simulink model "closedmodel"  (R2024b)
settings: Solver=ode4  StartTime=0.0  StopTime=10  FixedStep=0.001  RelTol=1e-3
values from neighbouring files (symbols this model uses):
  A = 0.00442    [closedparameters.m]
  Af = 0.003689    [closedparameters.m]
  alim = deg2rad(800)    [closedparameters.m]
  b = 0.14    [closedparameters.m]
  bt = 1    [closedparameters.m]
  Cd0 = 0.7    [closedparameters.m]
  Cla = 2    [closedparameters.m]
  Clp = -0.5    [closedparameters.m]
  Cmq = -40    [closedparameters.m]
  CNa = 20    [closedparameters.m]
  Cnr = -40    [closedparameters.m]
  Dgain = 0.2    [closedparameters.m]
  Dgainphi = 0.01    [closedparameters.m]
  dmdt = -(mf - me)/bt    (= -0.063)    [closedparameters.m]
  fin_positions = [dfins 0 fr; dfins -fr 0; dfins 0 -fr; dfins fr 0]    [closedparameters.m]
  gravity = [-9.819 0 0]'    [closedparameters.m]
  Igain = 0    [closedparameters.m]
  Igainphi = 0    [closedparameters.m]
  L = 1.15    [closedparameters.m]
  me = 0.894    [closedparameters.m]
  mf = 0.957    [closedparameters.m]
  N = [0 -1 0; 0 0 -1; 0 1 0; 0 0 1]    [closedparameters.m]
  Pgainphi = deg2rad(10)/ref_phi    [closedparameters.m]
  Pgainy = deg2rad(20)    [closedparameters.m]
  Pgainz = deg2rad(20)    [closedparameters.m]
  r_cp = [Cp 0 0]'    [closedparameters.m]
  ref_phi = pi/2    (= 1.57079632679)    [closedparameters.m]
  refy = 50    [closedparameters.m]
  refz = 50    [closedparameters.m]
  rho = 1.225    [closedparameters.m]
  si = [0 0 1; 0 -1 0; 0 0 -1; 0 1 0]    [closedparameters.m]
  tau = 0.05    [closedparameters.m]
  Vsafe = 0.1    [closedparameters.m]
  wind = [0 10 7]'    [closedparameters.m]
undefined symbols (not defined in the file or in its folder): fin_angles
libraries: slpidlib x5, aerolibanim x1, simulink x1, shared6dof x1, matrix_library x1
settings Model: Creator=tanel  LastModifiedBy=tanel
settings DataIOCC: ReturnWorkspaceOutputs=off

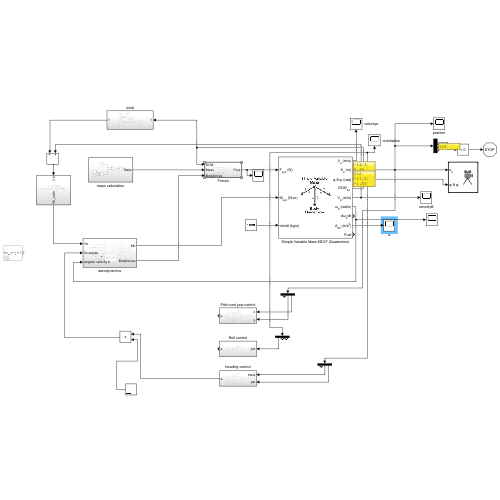
[thumbnail: Simulink's stored preview of the top-level diagram]
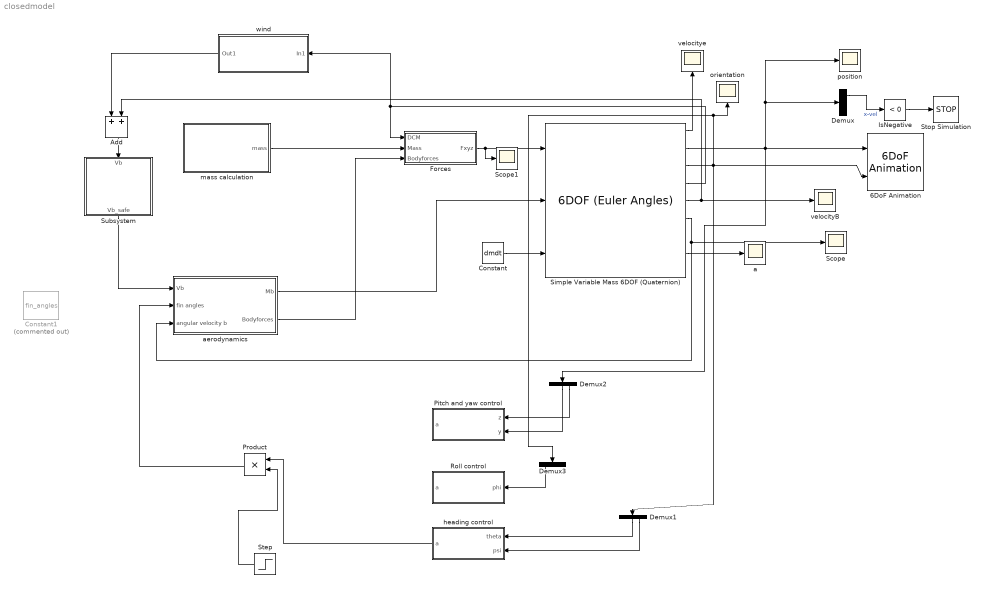
== system closedmodel ==
  6DoF Animation : aerolibanim/6DoF Animation  u1=[0 1000 0 100 0 100]  u2=0.01  u3=1  u4=[400 100 -500]  u5=Fly alongside  u6=[0 15 10]  u7=5  u8=on
  Add : Sum
  Constant : Constant  Value=dmdt
  Constant1 : Constant  Commented=on  Value=fin_angles
  Demux{,1..3} (4 alike) : Demux  Outputs=3
  Forces : Subsystem
  IsNegative : simulink/Logic and Bit Operations/Compare To Zero  relop=<  OutDataTypeStr=boolean
      settings: LibrarySourceBlock=|
      | simulink/Quick Insert/Logic and Bit
      | Operations/IsNegative
  Pitch and yaw control : Subsystem
  Product : Product
  Roll control : Subsystem
  Scope : Scope
  Scope1 : Scope
  Simple Variable Mass 6DOF (Quaternion) : shared6dof/6DOF (Euler Angles)  units=Metric (MKS)  mtype=Simple Variable  rep=Quaternion  xme_0=[0 50 50]  Vm_0=[0 0 0]  eul_0=[0 0 0]  pm_0=[0 0 0]  mass_0=mf  mass_e=me  mass_f=mf  inertia=eye(3)  inertia_e=Ie  inertia_f=If  k_quat=1.0  vre_flag=off  abi_flag=off  aMode=0  xme_statename=''  Vm_statename=''  eul_statename=''  quat_statename=''  pm_statename=''  mass_statename=''
      settings: LibrarySourceBlock=aerolib6dof2/Custom Variable Mass 6DOF (Euler Angles)
  Step : Step  SampleTime=0
  Stop Simulation : Stop
  Subsystem : Subsystem
  a : Scope
  aerodynamics : Subsystem
  heading control : Subsystem
  mass calculation : Subsystem
  orientation : Scope
  position : Scope
  velocityB : Scope
  velocitye : Scope
  wind : Subsystem
  wires:
  Constant/1 -> Simple Variable Mass 6DOF (Quaternion)/3
  Simple Variable Mass 6DOF (Quaternion)/4 -> wind/1(In1), Forces/1(DCM)
  Simple Variable Mass 6DOF (Quaternion)/5 -> Add/2, velocityB/1
  Forces/1(Fxyz) -> Scope1/1, Simple Variable Mass 6DOF (Quaternion)/1
  aerodynamics/1(Mb) -> Simple Variable Mass 6DOF (Quaternion)/2
  Simple Variable Mass 6DOF (Quaternion)/3 -> Demux1/1, 6DoF Animation/2, orientation/1, Demux3/1
  Simple Variable Mass 6DOF (Quaternion)/2 -> Demux/1, position/1, Demux2/1, 6DoF Animation/1
  IsNegative/1 -> Stop Simulation/1
  mass calculation/1(mass) -> Forces/2(Mass)
  Simple Variable Mass 6DOF (Quaternion)/1 -> velocitye/1
  Simple Variable Mass 6DOF (Quaternion)/8 -> a/1
  Simple Variable Mass 6DOF (Quaternion)/6 -> aerodynamics/3(angular velocity b), Scope/1
  aerodynamics/2(Bodyforces) -> Forces/3(Bodyforces)
  Subsystem/1(Vb_safe) -> aerodynamics/1(Vb)
  Demux2/2 -> Pitch and yaw control/2(y)
  Demux3/1 -> Roll control/1(phi)
  Demux2/3 -> Pitch and yaw control/1(z)
  Add/1 -> Subsystem/1(Vb)
  Step/1 -> Product/2
  Product/1 -> aerodynamics/2(fin angles)
  Demux1/2 -> heading control/1(theta)
  Demux1/3 -> heading control/2(psi)
  heading control/1(a) -> Product/1
  Demux/1 -> IsNegative/1  "x-vel"
  wind/1(Out1) -> Add/1

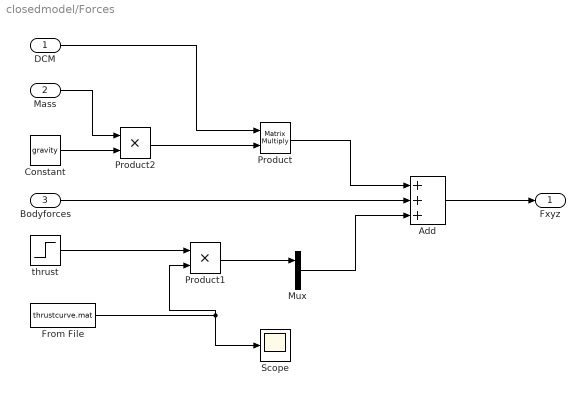
== system closedmodel/Forces ==
  DCM : Inport
  Mass : Inport  Port=2
  Bodyforces : Inport  Port=3
  Add : Sum  Inputs=+|+|+
  Constant : Constant  Value=gravity  VectorParams1D=off
  From File : FromFile  FileName=thrustcurve.mat  SampleTime=0
  Mux : Mux  Inputs=3
  Product : Product  Multiplication=Matrix(*)
  Product1 : Product
  Product2 : Product
  Scope : Scope
  thrust : Step  Time=bt  Before=1  After=0  SampleTime=0  VectorParams1D=off
  Fxyz : Outport
  wires:
  Add/1 -> Fxyz/1
  Constant/1 -> Product2/2
  Mass/1 -> Product2/1
  Product/1 -> Add/1
  DCM/1 -> Product/1
  Product2/1 -> Product/2
  Bodyforces/1 -> Add/2
  From File/1 -> Scope/1, Product1/2
  Mux/1 -> Add/3
  thrust/1 -> Product1/1
  Product1/1 -> Mux/1

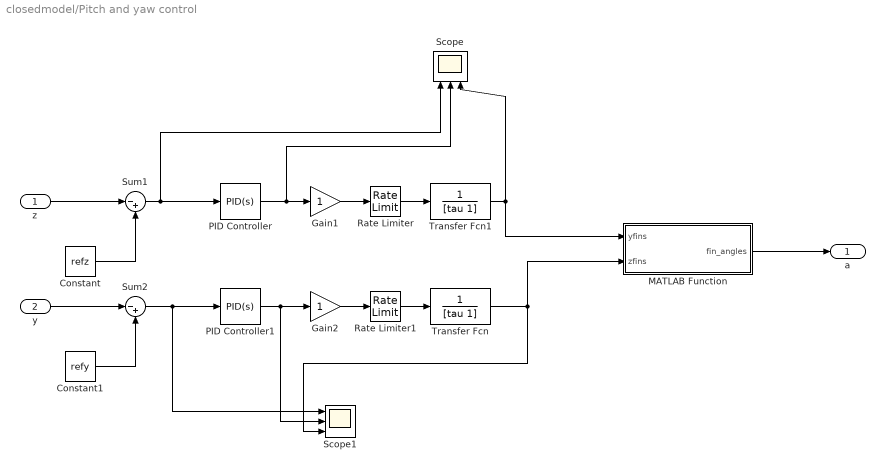
== system closedmodel/Pitch and yaw control ==
  z : Inport
  y : Inport  Port=2
  Constant : Constant  Value=refz
  Constant1 : Constant  Value=refy
  Gain1 : Gain
  Gain2 : Gain
  MATLAB Function : MATLAB Function  TreatAsAtomicUnit=on
  PID Controller : slpidlib/PID Controller  Controller=PID  Form=Parallel  TimeDomain=Continuous-time  UseExternalTs=off  SampleTime=-1  IntegratorMethod=Forward Euler  FilterMethod=Forward Euler  ControllerParametersSource=internal  P=Pgainz  I=Igain  UseKiTs=off  D=Dgain  UseExternalDerivativeSource=off  N=100  UseFilter=on  TunerSelectOption=Transfer Function Based (PID Tuner App)  InitialConditionSource=internal  InitialConditionForIntegrator=0  InitialConditionForFilter=0  DifferentiatorICPrevScaledInput=0  ExternalReset=none  TrackingMode=off  Kt=1  LimitOutput=on  SatLimitsSource=internal  UpperSaturationLimit=deg2rad(20)  LowerSaturationLimit=-deg2rad(20)  LinearizeAsGain=off  AntiWindupMode=clamping  Kb=1  LimitIntegrator=on  UpperIntegratorSaturationLimit=deg2rad(20)  LowerIntegratorSaturationLimit=-deg2rad(20)  POutMin=[]  POutMax=[]  IOutMin=[]  IOutMax=[]  DOutMin=[]  DOutMax=[]  NOutMin=[]  NOutMax=[]  SumOutMin=[]  SumOutMax=[]  SaturationOutMin=[]  SaturationOutMax=[]  PParamMin=[]  PParamMax=[]  IParamMin=[]  IParamMax=[]  DParamMin=[]  DParamMax=[]  NParamMin=[]  NParamMax=[]  KbParamMin=[]  KbParamMax=[]  KtParamMin=[]  KtParamMax=[]  KbOutMin=[]  KbOutMax=[]  KtOutMin=[]  KtOutMax=[]  IntegratorOutMin=[]  IntegratorOutMax=[]  FilterOutMin=[]  FilterOutMax=[]  SumI1OutMin=[]  SumI1OutMax=[]  SumI2OutMin=[]  SumI2OutMax=[]  SumI3OutMin=[]  SumI3OutMax=[]  SumI4OutMin=[]  SumI4OutMax=[]  SumDOutMin=[]  SumDOutMax=[]  DifferentiatorOutMin=[]  DifferentiatorOutMax=[]  FilterDiffOutCoefMin=[]  FilterDiffOutCoefMax=[]  ReciprocalOutMin=[]  ReciprocalOutMax=[]  SumDenOutMin=[]  SumDenOutMax=[]  SumNumOutMin=[]  SumNumOutMax=[]  DivideOutMin=[]  DivideOutMax=[]  UdiffTsProdOutMin=[]  UdiffTsProdOutMax=[]  NTsProdOutMin=[]  NTsProdOutMax=[]  UintegralTsProdOutMin=[]  UintegralTsProdOutMax=[]  UngainTsProdOutMin=[]  UngainTsProdOutMax=[]  ClampingZeroOutDataTypeStr=Inherit: Inherit via back propagation  ClampingZeroOutMin=[]  ClampingZeroOutMax=[]  FilterDenConstantOutDataTypeStr=Inherit: Inherit via back propagation  FilterDenConstantOutMin=[]  FilterDenConstantOutMax=[]  PCopyOutDataTypeStr=Inherit: Inherit via back propagation  PCopyOutMin=[]  PCopyOutMax=[]  NCopyOutDataTypeStr=Inherit: Inherit via back propagation  NCopyOutMin=[]  NCopyOutMax=[]  IntegratorContinuousStateAttributes=''  IntegratorStateMustResolveToSignalObject=off  IntegratorRTWStateStorageClass=Auto  FilterContinuousStateAttributes=''  FilterStateMustResolveToSignalObject=off  FilterRTWStateStorageClass=Auto  ParallelPVariant=InternalParameters  IdealPVariant=Disabled  IVariant=InternalParameters  DVariant=InternalParameters  IntegratorVariant=Continuous  SatVariant=Enabled  AWVariant=ContClampingParallel  PCopyVariant=Disabled  TRVariant=Disabled  FdbkBlocksVariant=Forward  IdealPFdbkVariant=Disabled  SatFdbkVariant=Disabled  DerivativeFilterVariant=ContFilter  NVariant=InternalParameters  NCopyVariant=Disabled  FilterICVariant=InternalICsFilter  IntegratorICVariant=InternalICs  ExternalResetVariant=Disabled  TRSumVariant=Passthrough  SumFdbkVariant=Disabled  SumVariant=Sum_PID  TsampFilterVariant=InternalTs  TsampNgainVariant=Passthrough  TsampIntegralVariant=Disabled_SignalSpec  ExternalSaturationOutDataTypeStr=Inherit: Same as second input  DerivativeSourceVariant=ErrorSignal  PreIntVariant=InternalPreInt
  PID Controller1 : slpidlib/PID Controller  Controller=PID  Form=Parallel  TimeDomain=Continuous-time  UseExternalTs=off  SampleTime=-1  IntegratorMethod=Forward Euler  FilterMethod=Forward Euler  ControllerParametersSource=internal  P=Pgainy  I=Igain  UseKiTs=off  D=Dgain  UseExternalDerivativeSource=off  N=100  UseFilter=on  TunerSelectOption=Transfer Function Based (PID Tuner App)  InitialConditionSource=internal  InitialConditionForIntegrator=0  InitialConditionForFilter=0  DifferentiatorICPrevScaledInput=0  ExternalReset=none  TrackingMode=off  Kt=1  LimitOutput=on  SatLimitsSource=internal  UpperSaturationLimit=deg2rad(20)  LowerSaturationLimit=-deg2rad(20)  LinearizeAsGain=on  AntiWindupMode=clamping  Kb=1  LimitIntegrator=on  UpperIntegratorSaturationLimit=deg2rad(20)  LowerIntegratorSaturationLimit=-deg2rad(20)  POutMin=[]  POutMax=[]  IOutMin=[]  IOutMax=[]  DOutMin=[]  DOutMax=[]  NOutMin=[]  NOutMax=[]  SumOutMin=[]  SumOutMax=[]  SaturationOutMin=[]  SaturationOutMax=[]  PParamMin=[]  PParamMax=[]  IParamMin=[]  IParamMax=[]  DParamMin=[]  DParamMax=[]  NParamMin=[]  NParamMax=[]  KbParamMin=[]  KbParamMax=[]  KtParamMin=[]  KtParamMax=[]  KbOutMin=[]  KbOutMax=[]  KtOutMin=[]  KtOutMax=[]  IntegratorOutMin=[]  IntegratorOutMax=[]  FilterOutMin=[]  FilterOutMax=[]  SumI1OutMin=[]  SumI1OutMax=[]  SumI2OutMin=[]  SumI2OutMax=[]  SumI3OutMin=[]  SumI3OutMax=[]  SumI4OutMin=[]  SumI4OutMax=[]  SumDOutMin=[]  SumDOutMax=[]  DifferentiatorOutMin=[]  DifferentiatorOutMax=[]  FilterDiffOutCoefMin=[]  FilterDiffOutCoefMax=[]  ReciprocalOutMin=[]  ReciprocalOutMax=[]  SumDenOutMin=[]  SumDenOutMax=[]  SumNumOutMin=[]  SumNumOutMax=[]  DivideOutMin=[]  DivideOutMax=[]  UdiffTsProdOutMin=[]  UdiffTsProdOutMax=[]  NTsProdOutMin=[]  NTsProdOutMax=[]  UintegralTsProdOutMin=[]  UintegralTsProdOutMax=[]  UngainTsProdOutMin=[]  UngainTsProdOutMax=[]  ClampingZeroOutDataTypeStr=Inherit: Inherit via back propagation  ClampingZeroOutMin=[]  ClampingZeroOutMax=[]  FilterDenConstantOutDataTypeStr=Inherit: Inherit via back propagation  FilterDenConstantOutMin=[]  FilterDenConstantOutMax=[]  PCopyOutDataTypeStr=Inherit: Inherit via back propagation  PCopyOutMin=[]  PCopyOutMax=[]  NCopyOutDataTypeStr=Inherit: Inherit via back propagation  NCopyOutMin=[]  NCopyOutMax=[]  IntegratorContinuousStateAttributes=''  IntegratorStateMustResolveToSignalObject=off  IntegratorRTWStateStorageClass=Auto  FilterContinuousStateAttributes=''  FilterStateMustResolveToSignalObject=off  FilterRTWStateStorageClass=Auto  ParallelPVariant=InternalParameters  IdealPVariant=Disabled  IVariant=InternalParameters  DVariant=InternalParameters  IntegratorVariant=Continuous  SatVariant=Enabled  AWVariant=ContClampingParallel  PCopyVariant=Disabled  TRVariant=Disabled  FdbkBlocksVariant=Forward  IdealPFdbkVariant=Disabled  SatFdbkVariant=Disabled  DerivativeFilterVariant=ContFilter  NVariant=InternalParameters  NCopyVariant=Disabled  FilterICVariant=InternalICsFilter  IntegratorICVariant=InternalICs  ExternalResetVariant=Disabled  TRSumVariant=Passthrough  SumFdbkVariant=Disabled  SumVariant=Sum_PID  TsampFilterVariant=InternalTs  TsampNgainVariant=Passthrough  TsampIntegralVariant=Disabled_SignalSpec  ExternalSaturationOutDataTypeStr=Inherit: Same as second input  DerivativeSourceVariant=ErrorSignal  PreIntVariant=InternalPreInt
  Rate Limiter : RateLimiter  RisingSlewLimit=alim  FallingSlewLimit=-alim  SampleTimeMode=inherited
  Rate Limiter1 : RateLimiter  RisingSlewLimit=alim  FallingSlewLimit=-alim  SampleTimeMode=inherited
  Scope : Scope  NumInputPorts=3
  Scope1 : Scope  NumInputPorts=3
  Sum1 : Sum  Inputs=|-+
  Sum2 : Sum  Inputs=|-+
  Transfer Fcn : TransferFcn  Denominator=[tau 1]
  Transfer Fcn1 : TransferFcn  Denominator=[tau 1]
  a : Outport  OutMin=[-deg2rad(15)]  OutMax=[deg2rad(15)]
  wires:
  Gain1/1 -> Rate Limiter/1
  z/1 -> Sum1/1
  Constant/1 -> Sum1/2
  Sum1/1 -> PID Controller/1, Scope/1
  PID Controller/1 -> Scope/2, Gain1/1
  y/1 -> Sum2/1
  Constant1/1 -> Sum2/2
  Sum2/1 -> Scope1/1, PID Controller1/1
  Gain2/1 -> Rate Limiter1/1
  PID Controller1/1 -> Gain2/1, Scope1/2
  MATLAB Function/1(fin_angles) -> a/1
  Rate Limiter/1 -> Transfer Fcn1/1
  Rate Limiter1/1 -> Transfer Fcn/1
  Transfer Fcn/1 -> MATLAB Function/2(zfins), Scope1/3
  Transfer Fcn1/1 -> MATLAB Function/1(yfins), Scope/3

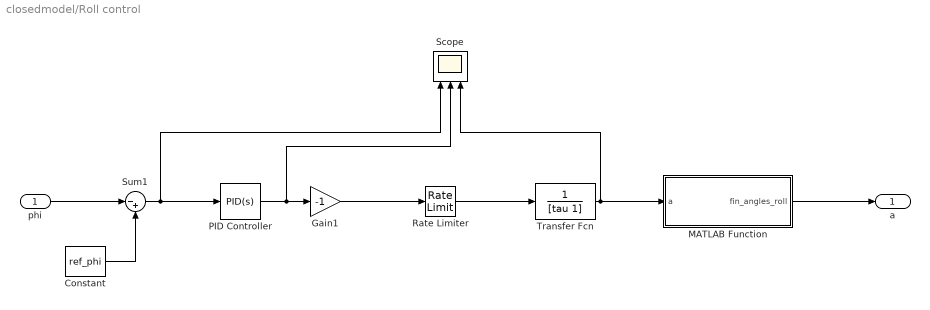
== system closedmodel/Roll control ==
  phi : Inport
  Constant : Constant  Value=ref_phi
  Gain1 : Gain  Gain=-1
  MATLAB Function : MATLAB Function  TreatAsAtomicUnit=on
  PID Controller : slpidlib/PID Controller  Controller=PID  Form=Parallel  TimeDomain=Continuous-time  UseExternalTs=off  SampleTime=-1  IntegratorMethod=Forward Euler  FilterMethod=Forward Euler  ControllerParametersSource=internal  P=Pgainphi  I=Igainphi  UseKiTs=off  D=Dgainphi  UseExternalDerivativeSource=off  N=100  UseFilter=on  TunerSelectOption=Transfer Function Based (PID Tuner App)  InitialConditionSource=internal  InitialConditionForIntegrator=0  InitialConditionForFilter=0  DifferentiatorICPrevScaledInput=0  ExternalReset=none  TrackingMode=off  Kt=1  LimitOutput=on  SatLimitsSource=internal  UpperSaturationLimit=deg2rad(20)  LowerSaturationLimit=-deg2rad(20)  LinearizeAsGain=on  AntiWindupMode=clamping  Kb=1  LimitIntegrator=on  UpperIntegratorSaturationLimit=deg2rad(20)  LowerIntegratorSaturationLimit=-deg2rad(20)  POutMin=[]  POutMax=[]  IOutMin=[]  IOutMax=[]  DOutMin=[]  DOutMax=[]  NOutMin=[]  NOutMax=[]  SumOutMin=[]  SumOutMax=[]  SaturationOutMin=[]  SaturationOutMax=[]  PParamMin=[]  PParamMax=[]  IParamMin=[]  IParamMax=[]  DParamMin=[]  DParamMax=[]  NParamMin=[]  NParamMax=[]  KbParamMin=[]  KbParamMax=[]  KtParamMin=[]  KtParamMax=[]  KbOutMin=[]  KbOutMax=[]  KtOutMin=[]  KtOutMax=[]  IntegratorOutMin=[]  IntegratorOutMax=[]  FilterOutMin=[]  FilterOutMax=[]  SumI1OutMin=[]  SumI1OutMax=[]  SumI2OutMin=[]  SumI2OutMax=[]  SumI3OutMin=[]  SumI3OutMax=[]  SumI4OutMin=[]  SumI4OutMax=[]  SumDOutMin=[]  SumDOutMax=[]  DifferentiatorOutMin=[]  DifferentiatorOutMax=[]  FilterDiffOutCoefMin=[]  FilterDiffOutCoefMax=[]  ReciprocalOutMin=[]  ReciprocalOutMax=[]  SumDenOutMin=[]  SumDenOutMax=[]  SumNumOutMin=[]  SumNumOutMax=[]  DivideOutMin=[]  DivideOutMax=[]  UdiffTsProdOutMin=[]  UdiffTsProdOutMax=[]  NTsProdOutMin=[]  NTsProdOutMax=[]  UintegralTsProdOutMin=[]  UintegralTsProdOutMax=[]  UngainTsProdOutMin=[]  UngainTsProdOutMax=[]  ClampingZeroOutDataTypeStr=Inherit: Inherit via back propagation  ClampingZeroOutMin=[]  ClampingZeroOutMax=[]  FilterDenConstantOutDataTypeStr=Inherit: Inherit via back propagation  FilterDenConstantOutMin=[]  FilterDenConstantOutMax=[]  PCopyOutDataTypeStr=Inherit: Inherit via back propagation  PCopyOutMin=[]  PCopyOutMax=[]  NCopyOutDataTypeStr=Inherit: Inherit via back propagation  NCopyOutMin=[]  NCopyOutMax=[]  IntegratorContinuousStateAttributes=''  IntegratorStateMustResolveToSignalObject=off  IntegratorRTWStateStorageClass=Auto  FilterContinuousStateAttributes=''  FilterStateMustResolveToSignalObject=off  FilterRTWStateStorageClass=Auto  ParallelPVariant=InternalParameters  IdealPVariant=Disabled  IVariant=InternalParameters  DVariant=InternalParameters  IntegratorVariant=Continuous  SatVariant=Enabled  AWVariant=ContClampingParallel  PCopyVariant=Disabled  TRVariant=Disabled  FdbkBlocksVariant=Forward  IdealPFdbkVariant=Disabled  SatFdbkVariant=Disabled  DerivativeFilterVariant=ContFilter  NVariant=InternalParameters  NCopyVariant=Disabled  FilterICVariant=InternalICsFilter  IntegratorICVariant=InternalICs  ExternalResetVariant=Disabled  TRSumVariant=Passthrough  SumFdbkVariant=Disabled  SumVariant=Sum_PID  TsampFilterVariant=InternalTs  TsampNgainVariant=Passthrough  TsampIntegralVariant=Disabled_SignalSpec  ExternalSaturationOutDataTypeStr=Inherit: Same as second input  DerivativeSourceVariant=ErrorSignal  PreIntVariant=InternalPreInt
  Rate Limiter : RateLimiter  RisingSlewLimit=alim  FallingSlewLimit=-alim  SampleTimeMode=inherited
  Scope : Scope  NumInputPorts=3
  Sum1 : Sum  Inputs=|-+
  Transfer Fcn : TransferFcn  Denominator=[tau 1]
  a : Outport  OutMin=[-deg2rad(15)]  OutMax=[deg2rad(15)]
  wires:
  Gain1/1 -> Rate Limiter/1
  phi/1 -> Sum1/1
  Constant/1 -> Sum1/2
  Sum1/1 -> PID Controller/1, Scope/1
  PID Controller/1 -> Scope/2, Gain1/1
  MATLAB Function/1(fin_angles_roll) -> a/1
  Rate Limiter/1 -> Transfer Fcn/1
  Transfer Fcn/1 -> Scope/3, MATLAB Function/1(a)

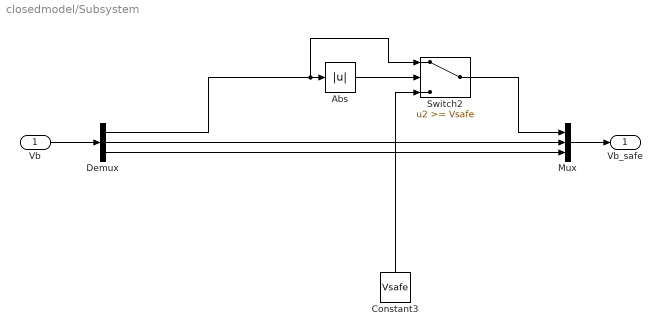
== system closedmodel/Subsystem ==
  Vb : Inport
  Abs : Abs  SaturateOnIntegerOverflow=off
  Constant3 : Constant  Value=Vsafe
  Demux : Demux  Outputs=3
  Mux : Mux  Inputs=3
  Switch2 : Switch  Threshold=Vsafe  SaturateOnIntegerOverflow=off  InputSameDT=off
  Vb_safe : Outport
  wires:
  Vb/1 -> Demux/1
  Abs/1 -> Switch2/2
  Demux/2 -> Mux/2
  Demux/3 -> Mux/3
  Switch2/1 -> Mux/1
  Mux/1 -> Vb_safe/1
  Demux/1 -> Switch2/1, Abs/1
  Constant3/1 -> Switch2/3

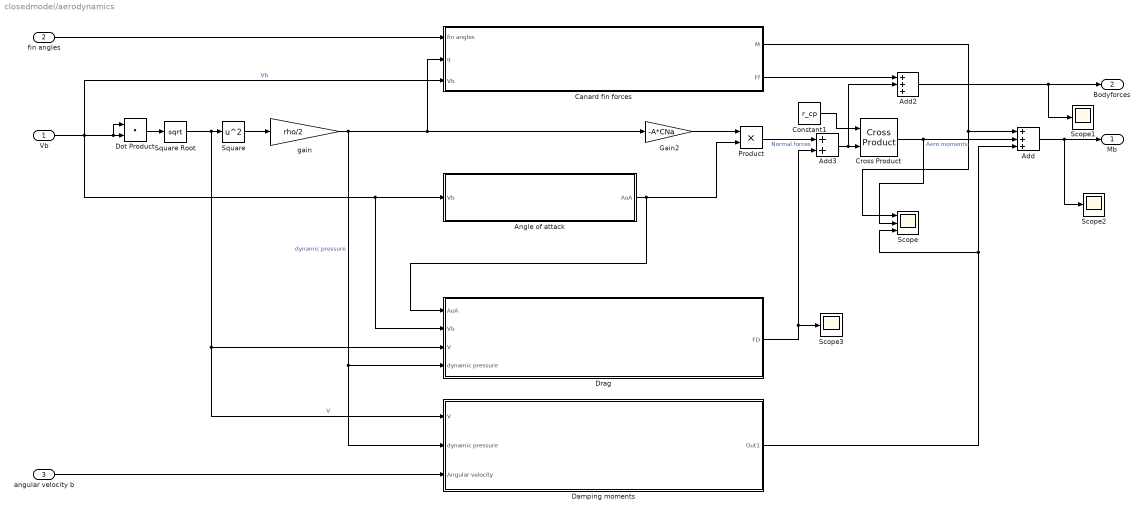
== system closedmodel/aerodynamics ==
  Vb : Inport
  fin angles : Inport  Port=2
  angular velocity b : Inport  Port=3
  Add : Sum  Inputs=+++
  Add2 : Sum  Inputs=+++
  Add3 : Sum
  Angle of attack : Subsystem
  Canard fin forces : Subsystem
  Constant1 : Constant  Value=r_cp
  Cross Product : matrix_library/Cross Product
  Damping moments : Subsystem
  Dot Product : DotProduct  OutDataTypeStr=Inherit: Inherit via internal rule
  Drag : Subsystem
  Gain2 : Gain  Gain=-A*CNa
  Product : Product
  Scope : Scope  NumInputPorts=3
  Scope1 : Scope
  Scope2 : Scope
  Scope3 : Scope
  Square : Math  Operator=square
  Square Root : Sqrt
  gain : Gain  Gain=rho/2
  Mb : Outport
  Bodyforces : Outport  Port=2
  wires:
  Gain2/1 -> Product/1
  Constant1/1 -> Cross Product/1
  Product/1 -> Add3/1  "Normal forces"
  Cross Product/1 -> Scope/2, Add/2  "Aero moments"
  Add/1 -> Scope2/1, Mb/1
  Add2/1 -> Scope1/1, Bodyforces/1
  Canard fin forces/2(Ff) -> Add2/1
  Add3/1 -> Add2/2, Cross Product/2
  Vb/1 -> Canard fin forces/3(Vb), Dot Product/1, Dot Product/2, Angle of attack/1(Vb), Drag/2(Vb)  "Vb"
  Square/1 -> gain/1
  Square Root/1 -> Damping moments/1(V), Drag/3(V), Square/1  "V"
  Dot Product/1 -> Square Root/1
  gain/1 -> Damping moments/2(dynamic pressure), Drag/4(dynamic pressure), Canard fin forces/2(q), Gain2/1  "dynamic pressure"
  fin angles/1 -> Canard fin forces/1(fin angles)
  Canard fin forces/1(M) -> Scope/1, Add/1
  Drag/1(FD) -> Scope3/1, Add3/2
  Angle of attack/1(AoA) -> Product/2, Drag/1(AoA)
  angular velocity b/1 -> Damping moments/3(Angular velocity)
  Damping moments/1(Out1) -> Add/3, Scope/3

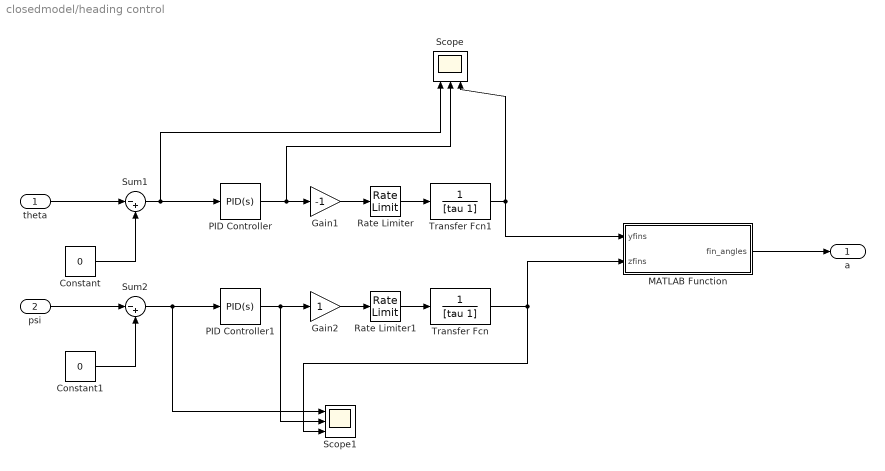
== system closedmodel/heading control ==
  theta : Inport
  psi : Inport  Port=2
  Constant : Constant  Value=0
  Constant1 : Constant  Value=0
  Gain1 : Gain  Gain=-1
  Gain2 : Gain
  MATLAB Function : MATLAB Function  TreatAsAtomicUnit=on
  PID Controller : slpidlib/PID Controller  Controller=PID  Form=Parallel  TimeDomain=Continuous-time  UseExternalTs=off  SampleTime=-1  IntegratorMethod=Forward Euler  FilterMethod=Forward Euler  ControllerParametersSource=internal  P=Pgainz  I=Igain  UseKiTs=off  D=Dgain  UseExternalDerivativeSource=off  N=100  UseFilter=on  TunerSelectOption=Transfer Function Based (PID Tuner App)  InitialConditionSource=internal  InitialConditionForIntegrator=0  InitialConditionForFilter=0  DifferentiatorICPrevScaledInput=0  ExternalReset=none  TrackingMode=off  Kt=1  LimitOutput=on  SatLimitsSource=internal  UpperSaturationLimit=deg2rad(20)  LowerSaturationLimit=-deg2rad(20)  LinearizeAsGain=off  AntiWindupMode=clamping  Kb=1  LimitIntegrator=on  UpperIntegratorSaturationLimit=deg2rad(20)  LowerIntegratorSaturationLimit=-deg2rad(20)  POutMin=[]  POutMax=[]  IOutMin=[]  IOutMax=[]  DOutMin=[]  DOutMax=[]  NOutMin=[]  NOutMax=[]  SumOutMin=[]  SumOutMax=[]  SaturationOutMin=[]  SaturationOutMax=[]  PParamMin=[]  PParamMax=[]  IParamMin=[]  IParamMax=[]  DParamMin=[]  DParamMax=[]  NParamMin=[]  NParamMax=[]  KbParamMin=[]  KbParamMax=[]  KtParamMin=[]  KtParamMax=[]  KbOutMin=[]  KbOutMax=[]  KtOutMin=[]  KtOutMax=[]  IntegratorOutMin=[]  IntegratorOutMax=[]  FilterOutMin=[]  FilterOutMax=[]  SumI1OutMin=[]  SumI1OutMax=[]  SumI2OutMin=[]  SumI2OutMax=[]  SumI3OutMin=[]  SumI3OutMax=[]  SumI4OutMin=[]  SumI4OutMax=[]  SumDOutMin=[]  SumDOutMax=[]  DifferentiatorOutMin=[]  DifferentiatorOutMax=[]  FilterDiffOutCoefMin=[]  FilterDiffOutCoefMax=[]  ReciprocalOutMin=[]  ReciprocalOutMax=[]  SumDenOutMin=[]  SumDenOutMax=[]  SumNumOutMin=[]  SumNumOutMax=[]  DivideOutMin=[]  DivideOutMax=[]  UdiffTsProdOutMin=[]  UdiffTsProdOutMax=[]  NTsProdOutMin=[]  NTsProdOutMax=[]  UintegralTsProdOutMin=[]  UintegralTsProdOutMax=[]  UngainTsProdOutMin=[]  UngainTsProdOutMax=[]  ClampingZeroOutDataTypeStr=Inherit: Inherit via back propagation  ClampingZeroOutMin=[]  ClampingZeroOutMax=[]  FilterDenConstantOutDataTypeStr=Inherit: Inherit via back propagation  FilterDenConstantOutMin=[]  FilterDenConstantOutMax=[]  PCopyOutDataTypeStr=Inherit: Inherit via back propagation  PCopyOutMin=[]  PCopyOutMax=[]  NCopyOutDataTypeStr=Inherit: Inherit via back propagation  NCopyOutMin=[]  NCopyOutMax=[]  IntegratorContinuousStateAttributes=''  IntegratorStateMustResolveToSignalObject=off  IntegratorRTWStateStorageClass=Auto  FilterContinuousStateAttributes=''  FilterStateMustResolveToSignalObject=off  FilterRTWStateStorageClass=Auto  ParallelPVariant=InternalParameters  IdealPVariant=Disabled  IVariant=InternalParameters  DVariant=InternalParameters  IntegratorVariant=Continuous  SatVariant=Enabled  AWVariant=ContClampingParallel  PCopyVariant=Disabled  TRVariant=Disabled  FdbkBlocksVariant=Forward  IdealPFdbkVariant=Disabled  SatFdbkVariant=Disabled  DerivativeFilterVariant=ContFilter  NVariant=InternalParameters  NCopyVariant=Disabled  FilterICVariant=InternalICsFilter  IntegratorICVariant=InternalICs  ExternalResetVariant=Disabled  TRSumVariant=Passthrough  SumFdbkVariant=Disabled  SumVariant=Sum_PID  TsampFilterVariant=InternalTs  TsampNgainVariant=Passthrough  TsampIntegralVariant=Disabled_SignalSpec  ExternalSaturationOutDataTypeStr=Inherit: Same as second input  DerivativeSourceVariant=ErrorSignal  PreIntVariant=InternalPreInt
  PID Controller1 : slpidlib/PID Controller  Controller=PID  Form=Parallel  TimeDomain=Continuous-time  UseExternalTs=off  SampleTime=-1  IntegratorMethod=Forward Euler  FilterMethod=Forward Euler  ControllerParametersSource=internal  P=Pgainy  I=Igain  UseKiTs=off  D=Dgain  UseExternalDerivativeSource=off  N=100  UseFilter=on  TunerSelectOption=Transfer Function Based (PID Tuner App)  InitialConditionSource=internal  InitialConditionForIntegrator=0  InitialConditionForFilter=0  DifferentiatorICPrevScaledInput=0  ExternalReset=none  TrackingMode=off  Kt=1  LimitOutput=on  SatLimitsSource=internal  UpperSaturationLimit=deg2rad(20)  LowerSaturationLimit=-deg2rad(20)  LinearizeAsGain=on  AntiWindupMode=clamping  Kb=1  LimitIntegrator=on  UpperIntegratorSaturationLimit=deg2rad(20)  LowerIntegratorSaturationLimit=-deg2rad(20)  POutMin=[]  POutMax=[]  IOutMin=[]  IOutMax=[]  DOutMin=[]  DOutMax=[]  NOutMin=[]  NOutMax=[]  SumOutMin=[]  SumOutMax=[]  SaturationOutMin=[]  SaturationOutMax=[]  PParamMin=[]  PParamMax=[]  IParamMin=[]  IParamMax=[]  DParamMin=[]  DParamMax=[]  NParamMin=[]  NParamMax=[]  KbParamMin=[]  KbParamMax=[]  KtParamMin=[]  KtParamMax=[]  KbOutMin=[]  KbOutMax=[]  KtOutMin=[]  KtOutMax=[]  IntegratorOutMin=[]  IntegratorOutMax=[]  FilterOutMin=[]  FilterOutMax=[]  SumI1OutMin=[]  SumI1OutMax=[]  SumI2OutMin=[]  SumI2OutMax=[]  SumI3OutMin=[]  SumI3OutMax=[]  SumI4OutMin=[]  SumI4OutMax=[]  SumDOutMin=[]  SumDOutMax=[]  DifferentiatorOutMin=[]  DifferentiatorOutMax=[]  FilterDiffOutCoefMin=[]  FilterDiffOutCoefMax=[]  ReciprocalOutMin=[]  ReciprocalOutMax=[]  SumDenOutMin=[]  SumDenOutMax=[]  SumNumOutMin=[]  SumNumOutMax=[]  DivideOutMin=[]  DivideOutMax=[]  UdiffTsProdOutMin=[]  UdiffTsProdOutMax=[]  NTsProdOutMin=[]  NTsProdOutMax=[]  UintegralTsProdOutMin=[]  UintegralTsProdOutMax=[]  UngainTsProdOutMin=[]  UngainTsProdOutMax=[]  ClampingZeroOutDataTypeStr=Inherit: Inherit via back propagation  ClampingZeroOutMin=[]  ClampingZeroOutMax=[]  FilterDenConstantOutDataTypeStr=Inherit: Inherit via back propagation  FilterDenConstantOutMin=[]  FilterDenConstantOutMax=[]  PCopyOutDataTypeStr=Inherit: Inherit via back propagation  PCopyOutMin=[]  PCopyOutMax=[]  NCopyOutDataTypeStr=Inherit: Inherit via back propagation  NCopyOutMin=[]  NCopyOutMax=[]  IntegratorContinuousStateAttributes=''  IntegratorStateMustResolveToSignalObject=off  IntegratorRTWStateStorageClass=Auto  FilterContinuousStateAttributes=''  FilterStateMustResolveToSignalObject=off  FilterRTWStateStorageClass=Auto  ParallelPVariant=InternalParameters  IdealPVariant=Disabled  IVariant=InternalParameters  DVariant=InternalParameters  IntegratorVariant=Continuous  SatVariant=Enabled  AWVariant=ContClampingParallel  PCopyVariant=Disabled  TRVariant=Disabled  FdbkBlocksVariant=Forward  IdealPFdbkVariant=Disabled  SatFdbkVariant=Disabled  DerivativeFilterVariant=ContFilter  NVariant=InternalParameters  NCopyVariant=Disabled  FilterICVariant=InternalICsFilter  IntegratorICVariant=InternalICs  ExternalResetVariant=Disabled  TRSumVariant=Passthrough  SumFdbkVariant=Disabled  SumVariant=Sum_PID  TsampFilterVariant=InternalTs  TsampNgainVariant=Passthrough  TsampIntegralVariant=Disabled_SignalSpec  ExternalSaturationOutDataTypeStr=Inherit: Same as second input  DerivativeSourceVariant=ErrorSignal  PreIntVariant=InternalPreInt
  Rate Limiter : RateLimiter  RisingSlewLimit=alim  FallingSlewLimit=-alim  SampleTimeMode=inherited
  Rate Limiter1 : RateLimiter  RisingSlewLimit=alim  FallingSlewLimit=-alim  SampleTimeMode=inherited
  Scope : Scope  NumInputPorts=3
  Scope1 : Scope  NumInputPorts=3
  Sum1 : Sum  Inputs=|-+
  Sum2 : Sum  Inputs=|-+
  Transfer Fcn : TransferFcn  Denominator=[tau 1]
  Transfer Fcn1 : TransferFcn  Denominator=[tau 1]
  a : Outport  OutMin=[-deg2rad(15)]  OutMax=[deg2rad(15)]
  wires:
  Gain1/1 -> Rate Limiter/1
  theta/1 -> Sum1/1
  Constant/1 -> Sum1/2
  Sum1/1 -> PID Controller/1, Scope/1
  PID Controller/1 -> Scope/2, Gain1/1
  psi/1 -> Sum2/1
  Constant1/1 -> Sum2/2
  Sum2/1 -> Scope1/1, PID Controller1/1
  Gain2/1 -> Rate Limiter1/1
  PID Controller1/1 -> Gain2/1, Scope1/2
  MATLAB Function/1(fin_angles) -> a/1
  Rate Limiter/1 -> Transfer Fcn1/1
  Rate Limiter1/1 -> Transfer Fcn/1
  Transfer Fcn/1 -> MATLAB Function/2(zfins), Scope1/3
  Transfer Fcn1/1 -> MATLAB Function/1(yfins), Scope/3

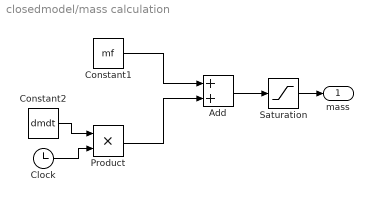
== system closedmodel/mass calculation ==
  Add : Sum  OutMin=me
  Clock : Clock
  Constant1 : Constant  Value=mf
  Constant2 : Constant  Value=dmdt
  Product : Product
  Saturation : Saturate  UpperLimit=mf  LowerLimit=me
  mass : Outport
  wires:
  Add/1 -> Saturation/1
  Constant1/1 -> Add/1
  Product/1 -> Add/2
  Clock/1 -> Product/2
  Saturation/1 -> mass/1
  Constant2/1 -> Product/1

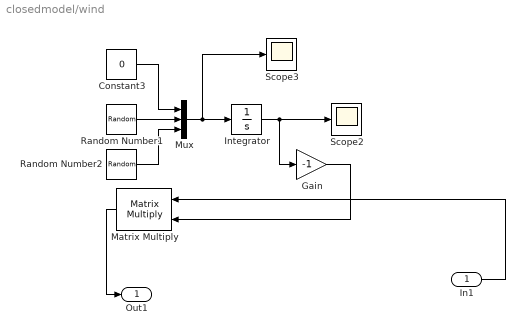
== system closedmodel/wind ==
  In1 : Inport
  Constant3 : Constant  Value=0
  Gain : Gain  Gain=-1
  Integrator : Integrator  InitialCondition=wind
  Matrix Multiply : Product  Multiplication=Matrix(*)
  Mux : Mux  Inputs=3
  Random Number1 : RandomNumber  Variance=2  Seed=randi(100)  SampleTime=0.01
  Random Number2 : RandomNumber  Variance=2  Seed=randi(100)  SampleTime=0.01
  Scope2 : Scope
  Scope3 : Scope
  Out1 : Outport
  wires:
  Mux/1 -> Scope3/1, Integrator/1
  Constant3/1 -> Mux/1
  Gain/1 -> Matrix Multiply/2
  Random Number1/1 -> Mux/2
  Random Number2/1 -> Mux/3
  Integrator/1 -> Gain/1, Scope2/1
  Matrix Multiply/1 -> Out1/1
  In1/1 -> Matrix Multiply/1

== system closedmodel/aerodynamics/Angle of attack ==
  Vb : Inport
  Atan : Trigonometry  Operator=atan
  Constant2 : Constant  Value=0
  Demux : Demux  Outputs=3
  Divide : Product  Inputs=/*  OutMin=[-pi]  OutMax=[pi]
  Mux : Mux  Inputs=3
  AoA : Outport
  wires:
  Mux/1 -> Divide/2
  Demux/2 -> Mux/2
  Demux/3 -> Mux/3
  Divide/1 -> Atan/1  "AoA (small a)"
  Constant2/1 -> Mux/1
  Atan/1 -> AoA/1  "AoA"
  Demux/1 -> Divide/1
  Vb/1 -> Demux/1

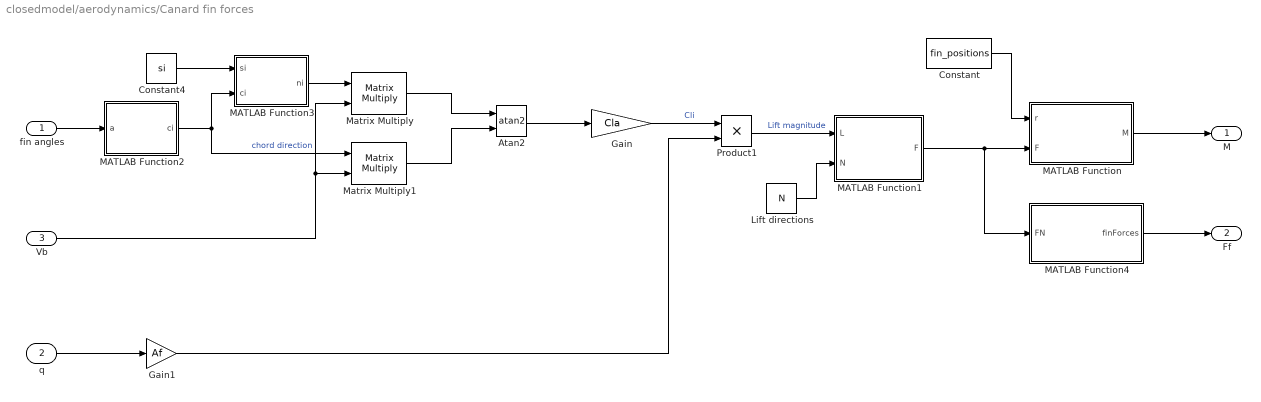
== system closedmodel/aerodynamics/Canard fin forces ==
  fin angles : Inport
  q : Inport  Port=2
  Vb : Inport  Port=3
  Atan2 : Trigonometry  Operator=atan2
  Constant : Constant  Value=fin_positions
  Constant4 : Constant  Value=si
  Gain : Gain  Gain=Cla
  Gain1 : Gain  Gain=Af
  Lift directions : Constant  Value=N
  MATLAB Function : MATLAB Function  TreatAsAtomicUnit=on
  MATLAB Function1 : MATLAB Function  TreatAsAtomicUnit=on
  MATLAB Function2 : MATLAB Function  TreatAsAtomicUnit=on
  MATLAB Function3 : MATLAB Function  TreatAsAtomicUnit=on
  MATLAB Function4 : MATLAB Function  TreatAsAtomicUnit=on
  Matrix Multiply : Product  Multiplication=Matrix(*)
  Matrix Multiply1 : Product  Multiplication=Matrix(*)
  Product1 : Product
  M : Outport
  Ff : Outport  Port=2
  wires:
  Constant4/1 -> MATLAB Function3/1(si)
  MATLAB Function1/1(F) -> MATLAB Function4/1(FN), MATLAB Function/2(F)
  Matrix Multiply/1 -> Atan2/1
  Atan2/1 -> Gain/1
  Constant/1 -> MATLAB Function/1(r)
  Lift directions/1 -> MATLAB Function1/2(N)
  Product1/1 -> MATLAB Function1/1(L)  "Lift magnitude"
  Gain/1 -> Product1/1  "Cli"
  MATLAB Function2/1(ci) -> MATLAB Function3/2(ci), Matrix Multiply1/1  "chord direction"
  Vb/1 -> Matrix Multiply/2, Matrix Multiply1/2
  Matrix Multiply1/1 -> Atan2/2
  fin angles/1 -> MATLAB Function2/1(a)
  MATLAB Function3/1(ni) -> Matrix Multiply/1
  MATLAB Function/1(M) -> M/1
  q/1 -> Gain1/1
  Gain1/1 -> Product1/2
  MATLAB Function4/1(finForces) -> Ff/1

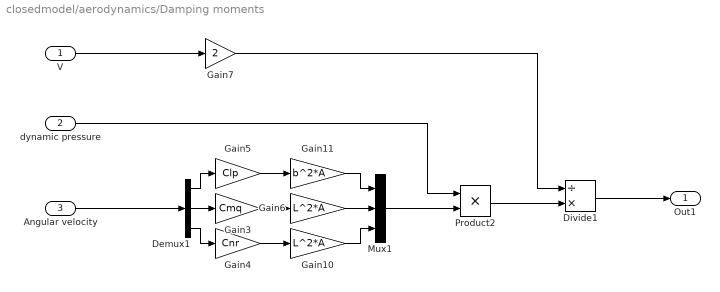
== system closedmodel/aerodynamics/Damping moments ==
  V : Inport
  dynamic pressure : Inport  Port=2
  Angular velocity : Inport  Port=3
  Demux1 : Demux  Outputs=3
  Divide1 : Product  Inputs=/*  SaturateOnIntegerOverflow=on
  Gain10 : Gain  Gain=L^2*A
  Gain11 : Gain  Gain=b^2*A
  Gain3 : Gain  Gain=Cmq
  Gain4 : Gain  Gain=Cnr
  Gain5 : Gain  Gain=Clp
  Gain6 : Gain  Gain=L^2*A
  Gain7 : Gain  Gain=2
  Mux1 : Mux  Inputs=3
  Product2 : Product
  Out1 : Outport
  wires:
  Mux1/1 -> Product2/2
  Gain11/1 -> Mux1/1
  Demux1/1 -> Gain5/1
  Demux1/2 -> Gain3/1
  Gain7/1 -> Divide1/1
  Product2/1 -> Divide1/2
  Demux1/3 -> Gain4/1
  Gain3/1 -> Gain6/1
  Gain5/1 -> Gain11/1
  Gain4/1 -> Gain10/1
  Gain10/1 -> Mux1/3
  Angular velocity/1 -> Demux1/1
  Gain6/1 -> Mux1/2
  Divide1/1 -> Out1/1
  V/1 -> Gain7/1
  dynamic pressure/1 -> Product2/1

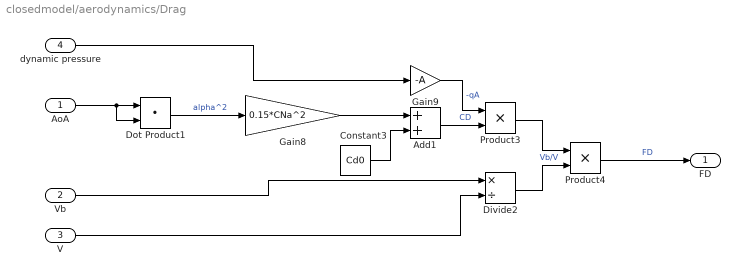
== system closedmodel/aerodynamics/Drag ==
  AoA : Inport
  Vb : Inport  Port=2
  V : Inport  Port=3
  dynamic pressure : Inport  Port=4
  Add1 : Sum
  Constant3 : Constant  Value=Cd0
  Divide2 : Product  Inputs=*/  SaturateOnIntegerOverflow=on
  Dot Product1 : DotProduct  OutDataTypeStr=Inherit: Inherit via internal rule
  Gain8 : Gain  Gain=0.15*CNa^2
  Gain9 : Gain  Gain=-A
  Product3 : Product
  Product4 : Product
  FD : Outport
  wires:
  AoA/1 -> Dot Product1/2, Dot Product1/1
  Product3/1 -> Product4/1
  Product4/1 -> FD/1  "FD"
  Vb/1 -> Divide2/1
  Divide2/1 -> Product4/2  "Vb/V"
  Constant3/1 -> Add1/2
  Add1/1 -> Product3/2  "CD"
  Gain9/1 -> Product3/1  "-qA"
  Gain8/1 -> Add1/1
  Dot Product1/1 -> Gain8/1  "alpha^2"
  dynamic pressure/1 -> Gain9/1
  V/1 -> Divide2/2

== matlab function closedmodel/aerodynamics/Canard fin forces/MATLAB Function1 ==
  data: L input; F output; N input
function F = scaleForces(L,N)

F = L .* N;

end

== matlab function closedmodel/aerodynamics/Canard fin forces/MATLAB Function ==
  data: r input; M output; F input
function M = computeTorque(r,F)

M = [0 0 0];

for i = 1:4
    M = M + cross(r(i,:), F(i,:));
end

end

== matlab function closedmodel/aerodynamics/Canard fin forces/MATLAB Function2 ==
  data: a input; ci output
function ci = chordDirections(a)
    ci = [cos(a(1)) sin(a(1)) 0; cos(a(2)) 0 sin(a(2)); cos(a(3)) -sin(a(3)) 0; cos(a(4)) 0 -sin(a(4))];
end

== matlab function closedmodel/Pitch and yaw control/MATLAB Function ==
  data: yfins input; zfins input; fin_angles output
function fin_angles = finangles(yfins, zfins)
    fin_angles = [zfins yfins -zfins -yfins]';
end

== matlab function closedmodel/aerodynamics/Canard fin forces/MATLAB Function3 ==
  data: si input; ni output; ci input
function ni = fcn(si, ci)
    ni = cross(si, ci);
end

== matlab function closedmodel/aerodynamics/Canard fin forces/MATLAB Function4 ==
  data: FN input; finForces output
function finForces = fcn(FN)
    finForces = sum(FN,1)';
end

== matlab function closedmodel/Roll control/MATLAB Function ==
  data: a input; fin_angles_roll output
function fin_angles_roll = finangles_roll(a)
    fin_angles_roll = [a a a a]';
end

== matlab function closedmodel/heading control/MATLAB Function ==
  data: yfins input; zfins input; fin_angles output
function fin_angles = finangles(yfins, zfins)
    fin_angles = [zfins yfins -zfins -yfins]';
end
